simulink model "Fsbb_simulink"  (R2024a)
settings: Solver=VariableStepAuto  StartTime=0.0  StopTime=100  RelTol=1e-3
libraries: spsSeriesRLCBranchLib x5, spsMosfetLib x4, spsCurrentMeasurementLib x1, spsDCVoltageSourceLib x1, spsVoltageMeasurementLib x1, sps_lib x1
settings Model: Creator=Victus  LastModifiedBy=Victus

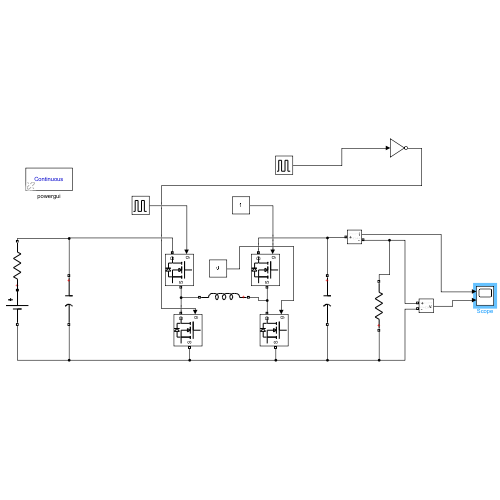
[thumbnail: Simulink's stored preview of the top-level diagram]
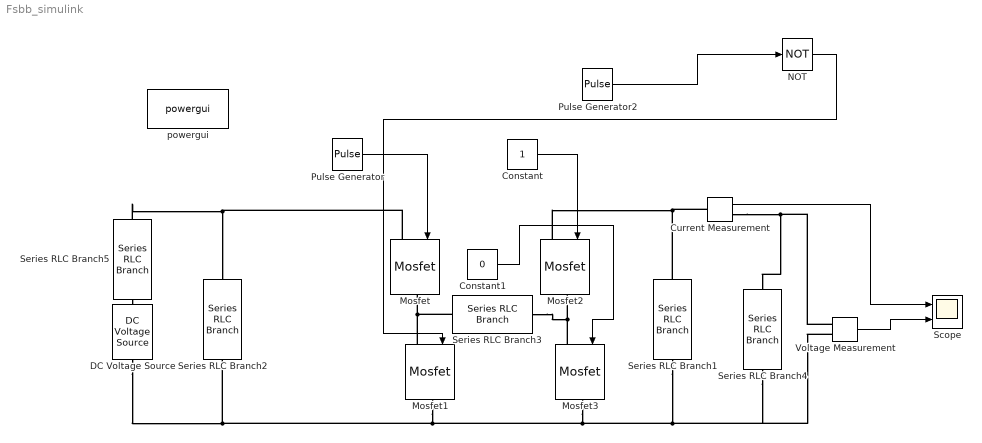
== system Fsbb_simulink ==
  Constant : Constant
  Constant1 : Constant  Value=0
  Current Measurement : spsCurrentMeasurementLib/Current Measurement  PhasorSimulation=off  OutputType=Complex  PSBequivalent=0
  DC Voltage Source : spsDCVoltageSourceLib/DC Voltage Source  Amplitude=20  Measurements=None
  Mosfet{,1..3} (4 alike) : spsMosfetLib/Mosfet  Ron=0.1  Lon=0  Rd=0.01  Vfd=0  IC=0  Rs=1e5  Cs=inf  Measurements=off
  NOT : Logic  Operator=NOT  IconShape=distinctive  AllPortsSameDT=off  OutDataTypeStr=boolean
  Pulse Generator : DiscretePulseGenerator  PulseType=Time based  Period=4e-05  PulseWidth=50  VectorParams1D=off
  Pulse Generator2 : DiscretePulseGenerator  PulseType=Time based  Period=4e-05  PulseWidth=50  VectorParams1D=off
  Scope : Scope  NumInputPorts=2
  Series RLC Branch1 : spsSeriesRLCBranchLib/Series RLC Branch  LConnTagsString=__new0  RConnTagsString=__new0  BranchType=C  Resistance=1  Inductance=1e-3  SetiL0=off  InitialCurrent=0  Capacitance=0.1  Setx0=off  InitialVoltage=0  Measurements=None
  Series RLC Branch2 : spsSeriesRLCBranchLib/Series RLC Branch  LConnTagsString=__new0  RConnTagsString=__new0  BranchType=C  Resistance=1  Inductance=1e-3  SetiL0=off  InitialCurrent=0  Capacitance=0.1  Setx0=off  InitialVoltage=0  Measurements=None
  Series RLC Branch3 : spsSeriesRLCBranchLib/Series RLC Branch  LConnTagsString=__new0  RConnTagsString=__new0  BranchType=L  Resistance=1  Inductance=0.1  SetiL0=off  InitialCurrent=0  Capacitance=1e-6  Setx0=off  InitialVoltage=0  Measurements=None
  Series RLC Branch4 : spsSeriesRLCBranchLib/Series RLC Branch  LConnTagsString=__new0  RConnTagsString=__new0  BranchType=R  Resistance=2  Inductance=1e-3  SetiL0=off  InitialCurrent=0  Capacitance=1e-6  Setx0=off  InitialVoltage=0  Measurements=None
  Series RLC Branch5 : spsSeriesRLCBranchLib/Series RLC Branch  LConnTagsString=__new0  RConnTagsString=__new0  BranchType=R  Resistance=0.0001  Inductance=1e-3  SetiL0=off  InitialCurrent=0  Capacitance=1e-6  Setx0=off  InitialVoltage=0  Measurements=None
  Voltage Measurement : spsVoltageMeasurementLib/Voltage Measurement  PhasorSimulation=off  OutputType=Complex  PSBequivalent=0
  powergui : sps_lib/powergui  Priority=1  SimulationMode=Continuous  SampleTime=50e-6  frequency=60  Iterations=50  frequencyindice=0  Pbase=100e6  ErrMax=1e-4  UnitsV=kV  UnitsW=MW  buscounter=0  FunctionMessages=off  echomessages=off  EnableUseOfTLC=off  CurrentSourceSwitches=off  DisableSnubberDevices=off  DisableRonSwitches=off  DisableVfSwitches=off  DisplayEquations=off  AutomaticDiscreteSolvers=off  SolverType=Tustin/Backward Euler (TBE)  Interpol=off  ExternalGateDelay=off  methode=off  Ts=100  x0status=blocks  SPID=on  SwTol=0  HookPort=off  NonlinearTolerance=1e-4  nMaxIteration=100  ContinueOnMaxIteration=off  RestoreLinks=warning  ResistiveCurrentMeasurement=off  Frange=[0:2:500]  Ylog=off  Xlog=on  ShowGrid=off  save=off  variable=ZData  structure=0  ZoomFFT=off  StartTime=0.0  cycles=1  DisplayStyle=1  fundamental=60  FreqAxis=off  MaxFrequency=1000  frequencyindicesteady=1  RmsSteady=1  display=off
  wires:
  Pulse Generator/1 -> Mosfet/1
  NOT/1 -> Mosfet1/1
  Constant/1 -> Mosfet2/1
  Voltage Measurement/1 -> Scope/2
  Current Measurement/1 -> Scope/1
  Constant1/1 -> Mosfet3/1
  Pulse Generator2/1 -> NOT/1
  connections:
  Mosfet2/LConn1 -- Series RLC Branch1/LConn1 -- Current Measurement/LConn1
  Mosfet1/LConn1 -- Series RLC Branch3/RConn1 -- Mosfet/RConn1
  DC Voltage Source/LConn1 -- Mosfet3/RConn1 -- Voltage Measurement/LConn2 -- Series RLC Branch4/LConn1 -- Series RLC Branch1/RConn1 -- Mosfet1/RConn1 -- Series RLC Branch2/RConn1
  Voltage Measurement/LConn1 -- Current Measurement/RConn1 -- Series RLC Branch4/RConn1
  Series RLC Branch3/LConn1 -- Mosfet3/LConn1 -- Mosfet2/RConn1
  Series RLC Branch5/LConn1 -- DC Voltage Source/RConn1
  Series RLC Branch5/RConn1 -- Mosfet/LConn1 -- Series RLC Branch2/LConn1
